simulink model "Vejlupek_CAR4_dsPIC33_AxleControl_bckup_R091228_R02"  (Simulink 7.3)
settings: Solver=FixedStepDiscrete  StartTime=0.0  StopTime=10.0  FixedStep=0.001  RelTol=1e-3
libraries: dsPICdrivers x14
settings Model: Creator=Bobes  LastModifiedBy=Bobes
settings OptimizationCC: OptimizeModelRefInitCode=on  LifeSpan=1
settings HardwareCC: ProdBitPerInt=16  ProdEndianess=LittleEndian  ProdWordSize=16  ProdHWDeviceType=16-bit Generic
settings RTWCC: SystemTargetFile=dspic.tlc  TemplateMakefile=dspic_pic30_gcc.tmf  PostCodeGenCommand=dsPIC_Compile()  Description=Embedded Target for Microchip dsPIC (real-time)  ProcessScript=dspic_make_rtw_hook
settings CodeAppCC: IgnoreCustomStorageClasses=off
settings STFCustomTargetCC: ModelReferenceCompliant=off  IncludeMdlTerminateFcn=off  CombineOutputUpdateFcns=on  SuppressErrorStatus=on  ERTCustomFileBanners=on  SupportContinuousTime=off  SupportNonInlinedSFcns=off  SystemTargetFile=dspic.tlc
settings ERTTargetCC: MultiwordLength=2048  ModelReferenceCompliant=off  ParMdlRefBuildCompliant=off  CompOptLevelCompliant=off  IncludeMdlTerminateFcn=off  SuppressErrorStatus=on  ERTFirstTimeCompliant=off  ModelStepFunctionPrototypeControlCompliant=off  CPPClassGenCompliant=off  InlinedParameterPlacement=NonHierarchical  ERTSrcFileBannerTemplate=dsPIC_code_template.cgt  ERTHdrFileBannerTemplate=dsPIC_code_template.cgt  ERTDataSrcFileTemplate=dsPIC_code_template.cgt  ERTDataHdrFileTemplate=dsPIC_code_template.cgt  ERTCustomFileTemplate=dsPIC_main.tlc
settings CustomProperty: DataType=string  Value=C:\PROGRA~1\MATLAB\R2009a\bin\win32\gmake

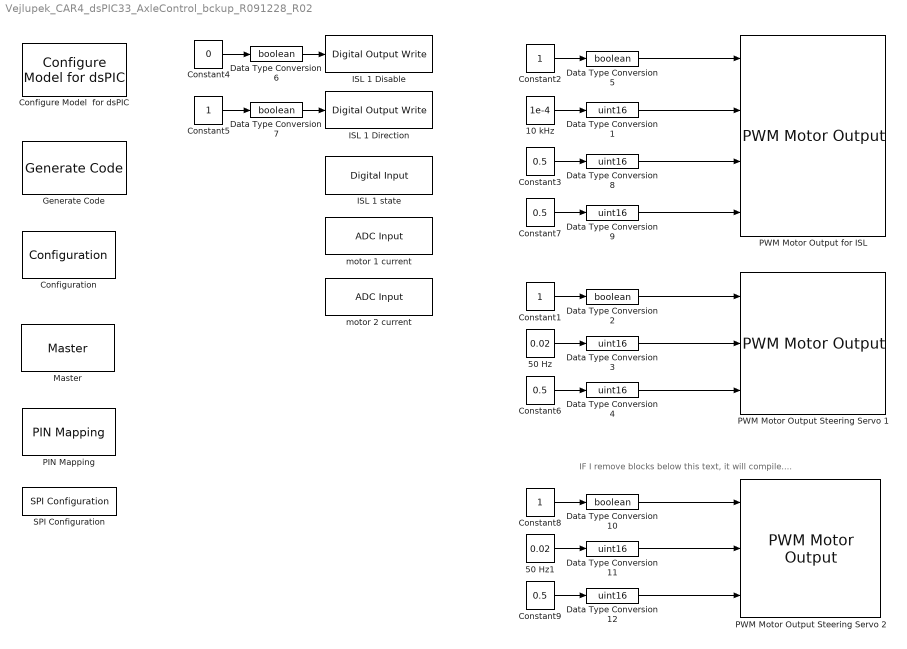
== system Vejlupek_CAR4_dsPIC33_AxleControl_bckup_R091228_R02 ==
  note: IF I remove blocks below this text, it will compile....
  10 kHz : Constant  Value=1e-4  OutDataType=fixdt(1, 16)  OutScaling=2^0
  50 Hz : Constant  Value=0.02  OutDataType=fixdt(1, 16)  OutScaling=2^0
  50 Hz1 : Constant  Value=0.02  OutDataType=fixdt(1, 16)  OutScaling=2^0
  Configuration : dsPICdrivers/Configuration  SystemSampleTime=-1  double64=on
  Configure Model  for dsPIC : dsPICdrivers/Simulink Configuration/Configure Model  for dsPIC
  Constant1 : Constant  OutDataType=fixdt(1, 16)  OutScaling=2^0
  Constant2 : Constant  OutDataType=fixdt(1, 16)  OutScaling=2^0
  Constant{3,6..7,9} (4 alike) : Constant  Value=0.5  OutDataType=fixdt(1, 16)  OutScaling=2^0
  Constant4 : Constant  Value=0  OutDataTypeMode=boolean  OutDataType=fixdt(1, 16)  OutScaling=2^0  OutDataTypeStr=boolean
  Constant5 : Constant  OutDataTypeMode=boolean  OutDataType=fixdt(1, 16)  OutScaling=2^0  OutDataTypeStr=boolean
  Constant8 : Constant  OutDataType=fixdt(1, 16)  OutScaling=2^0
  Data Type Conversion{1,3..4,8..9,11..12} (7 alike) : DataTypeConversion  OutDataTypeMode=uint16  OutDataType=fixdt(1, 16)  OutScaling=2^0  OutDataTypeStr=uint16
  Data Type Conversion{2,5..7,10} (5 alike) : DataTypeConversion  OutDataTypeMode=boolean  OutDataType=fixdt(1, 16)  OutScaling=2^0  OutDataTypeStr=boolean
  Generate Code : dsPICdrivers/Simulink Configuration/Generate Code
  ISL 1 Direction : dsPICdrivers/Digital I//O/Digital Output Write  Tag=dsPIC_Digital_Output  Priority=5  PORT=B  Pin=[4]  Simultaneous=off  OrderingInOutPopup=None
  ISL 1 Disable : dsPICdrivers/Digital I//O/Digital Output Write  Tag=dsPIC_Digital_Output  Priority=5  PORT=B  Pin=[3]  Simultaneous=off  OrderingInOutPopup=None
  ISL 1 state : dsPICdrivers/Digital I//O/Digital Input  Tag=dsPIC_Digital_Input  PORT=B  Pin=[2]  SampleTime=-1  OrderingInOutPopup=None
  Master : dsPICdrivers/Master  Tag=dsPIC_MASTER  Priority=1  TimeStepType=Timer1  picType=33fj128MC802  fcy=20000000  Quartz_33f=40e6  PLLActive_33f=off  fcyDesired_33f=20e6  tmr1="[1  19999  0]"  tmr1Info="Time Step : 0.001  ;   Error : 0%  PR1=19999"  tmr2345="[0  0  0  0]"  tmr2345cfg=[-1 -1 -1 -1]  IOautoConf=on  typePort="[ 8   8   0   0   0   0   0   0   0   0   0   0   0   0   0   0  22  22   9  10  10   0   0   0   0   0   0   0   0   0   0   0   0   0   0   0   0   0   0   0   0   0   0   0   0   0   0   0   0   0   0   0   0   0   0   0   0   0   0   0   0   0   0   0   0   0   0   0   0   0   0   0   0   0   0   0   0   0   0   0   0   0   0   0   0   0   0   0   0   0   0   0   0   0   0   0   0   0   0   0   0   0   0   0   0   0   0   0   0   0   0   0 ]"  TRIS="[ 65535  65511  65535  65535  65535  65535  65535 ]"  ADPCFG=60  MasterBusyPort=None  MasterOverloadPort=None  FOSC=External Clock  ClockSwitchMonitor=Both disabled  TempProtection_33f=TEMP_ON  FPBOR=<empty>  PWRT=disable  MCLR=<empty>  PowerSave=off  OverrideFcy=off  NewFcy=1e6  PR2345="[65535  65535  65535  65535]"
  PIN Mapping : dsPICdrivers/Peripheral MAPPING/PIN Mapping  Tag=dsPIC_PIN_Mapping  in_INT1=Not tied (VSS)  in_INT2=Not tied (VSS)  in_T2CK=Not tied (VSS)  in_T3CK=Not tied (VSS)  in_T4CK=Not tied (VSS)  in_T5CK=Not tied (VSS)  in_IC1=Not tied (VSS)  in_IC2=Not tied (VSS)  in_IC7=Not tied (VSS)  in_IC8=Not tied (VSS)  out_OC1=Not changed  out_OC2=Not changed  out_OC3=Not changed  out_OC4=Not changed  in_OCFA=Not tied (VSS)  in_FLTA1=Not tied (VSS)  in_FLTA2=Not tied (VSS)  in_QEA1=tied to RP0  in_QEB1=tied to RP1  in_INDX1=Not tied (VSS)  out_UPDN1=Not changed  out_UPDN2=Not changed  in_QEA2=Not changed  in_QEB2=Not changed  in_INDX2=Not tied (VSS)  in_U1RX=Not tied (VSS)  out_U1TX=Not changed  in_U1CTS=Not tied (VSS)  out_U1RTS=Not changed  in_U2RX=Not tied (VSS)  out_U2TX=Not changed  in_U2CTS=Not tied (VSS)  out_U2RTS=Not changed  in_SDI1=Not tied (VSS)  out_SDO1=Not changed  in_SCK1=Not tied (VSS)  out_SCK1OUT=Not changed  in_SS1=Not tied (VSS)  out_SS1OUT=Not changed  in_SDI2=Not tied (VSS)  out_SDO2=Not changed  in_SCK2=Not tied (VSS)  out_SCK2OUT=Not changed  in_SS2=Not tied (VSS)  out_SS2OUT=Not changed  in_C1RX=Not changed  out_C1TX=Not changed  out_C1OUT=Not changed  out_C2OUT=Not changed
  PWM Motor Output Steering Servo 1 : dsPICdrivers/Peripheral I//O/PWM Motor Output  Tag=dsPIC_PWM_Motor  Priority=5  PWMref=1  PWM12=2  InputEnableChk=on  InputPeriodeChk=on  Channel=[3]  TPeriode=0.02  PrescalerValue=16  PeriodeInteger=25000  MaxName='PWM'  Centered=off  HChannelON=off  Info="Nbr Bits : 15.6096  ||  PWM = 50000  ||  Prescaler = 16"  Delay=0  IntPriority=5  nbrPwmChannelPIC=3  Status=OK  DeadTimePrescaleA=0  DeadTimePrescaleB=0  DeadTimeInfo="Dead Time A = 0  ||  Dead Time B = 0"  DTPWM1a=Prescaler A  DTPWM1i=Prescaler A  DTPWM2a=Prescaler A  DTPWM2i=Prescaler A  DTPWM3a=Prescaler A  DTPWM3i=Prescaler A  DTPWM4a=Prescaler A  DTPWM4i=Prescaler A  DTCON1=0  DTCON2=0
  PWM Motor Output Steering Servo 2 : dsPICdrivers/Peripheral I//O/PWM Motor Output  Tag=dsPIC_PWM_Motor  Priority=5  PWMref=2  PWM12=2  InputEnableChk=on  InputPeriodeChk=on  Channel=[1]  TPeriode=.02  PrescalerValue=16  PeriodeInteger=25000  MaxName='PWM'  Centered=off  HChannelON=off  Info="Nbr Bits : 15.6096  ||  PWM = 50000  ||  Prescaler = 16"  Delay=0  IntPriority=5  nbrPwmChannelPIC=1  Status=OK  DeadTimePrescaleA=0  DeadTimePrescaleB=0  DeadTimeInfo="Dead Time A = 0  ||  Dead Time B = 0"  DTPWM1a=Prescaler A  DTPWM1i=Prescaler A  DTPWM2a=Prescaler A  DTPWM2i=Prescaler A  DTPWM3a=Prescaler A  DTPWM3i=Prescaler A  DTPWM4a=Prescaler A  DTPWM4i=Prescaler A  DTCON1=0  DTCON2=0
  PWM Motor Output for ISL : dsPICdrivers/Peripheral I//O/PWM Motor Output  Tag=dsPIC_PWM_Motor  Priority=5  PWMref=1  PWM12=2  InputEnableChk=on  InputPeriodeChk=on  Channel=[1 2]  TPeriode=1e-5  PrescalerValue=1  PeriodeInteger=200  MaxName='PWM'  Centered=off  HChannelON=off  Info="Nbr Bits : 8.6439  ||  PWM = 400  ||  Prescaler = 1"  Delay=0  IntPriority=5  nbrPwmChannelPIC=3  Status=OK  DeadTimePrescaleA=0  DeadTimePrescaleB=0  DeadTimeInfo="Dead Time A = 0  ||  Dead Time B = 0"  DTPWM1a=Prescaler A  DTPWM1i=Prescaler A  DTPWM2a=Prescaler A  DTPWM2i=Prescaler A  DTPWM3a=Prescaler A  DTPWM3i=Prescaler A  DTPWM4a=Prescaler A  DTPWM4i=Prescaler A  DTCON1=0  DTCON2=0
  SPI Configuration : dsPICdrivers/SPI PORT/SPI Configuration  Tag=dsPIC_config_SPI  Priority=2  ConfigurationTime=At boot time (only once)  OrderingInOutPopup=None  SampleTime=-1  Frame_Enable=0  Frame_Sync=None  SPI=1  MODE=MASTER  USER_SCALER=20  StartEnable=Enable  SDO_EN=off  DATA_LENGTH=16 bits  SS_EN=off  SMP=End of bit  CKP=high  CKE=Idle to Active  Status="OK - Mode 1  -    Fsck= 1000000Hz"
  motor 1 current : dsPICdrivers/Peripheral I//O/ADC Input  Tag=dsPIC_ADC  Priority=5  ADC_TYPE=10 bits  ADC_MODE=Continuous sampling & get last channel value  NbrSampleStep=1  VoltRefpopup="AVdd  -  AVss"  OutFormatBitspopup=0000 00dd dddd dddd : Integer  InterruptPriority=6  ANCHANNELS=[0]  MaxName=ANmax = 1023  Rin=1e2  ADCS=6  SAMC=1  Temperature=25  DMAChannel=0  SampleTime=-1  Status="OK  |  Tsmp=1.750e-007 |  T/Channel=2.275e-006 |  Tall=2.275e-006"  SSRC=auto convert
  motor 2 current : dsPICdrivers/Peripheral I//O/ADC Input  Tag=dsPIC_ADC  Priority=5  ADC_TYPE=10 bits  ADC_MODE=Continuous sampling & get last channel value  NbrSampleStep=1  VoltRefpopup="AVdd  -  AVss"  OutFormatBitspopup=0000 00dd dddd dddd : Integer  InterruptPriority=6  ANCHANNELS=[1]  MaxName=ANmax = 1023  Rin=1e2  ADCS=6  SAMC=1  Temperature=25  DMAChannel=0  SampleTime=-1  Status="OK  |  Tsmp=1.750e-007 |  T/Channel=2.275e-006 |  Tall=2.275e-006"  SSRC=auto convert
  wires:
  Constant2/1 -> Data Type Conversion5/1
  Data Type Conversion5/1 -> PWM Motor Output for ISL/1
  Constant1/1 -> Data Type Conversion2/1
  Data Type Conversion2/1 -> PWM Motor Output Steering Servo 1/1
  Data Type Conversion3/1 -> PWM Motor Output Steering Servo 1/2
  Data Type Conversion4/1 -> PWM Motor Output Steering Servo 1/3
  10 kHz/1 -> Data Type Conversion1/1
  Data Type Conversion1/1 -> PWM Motor Output for ISL/2
  50 Hz/1 -> Data Type Conversion3/1
  Constant6/1 -> Data Type Conversion4/1
  Constant5/1 -> Data Type Conversion7/1
  Data Type Conversion7/1 -> ISL 1 Direction/1
  Constant4/1 -> Data Type Conversion6/1
  Data Type Conversion6/1 -> ISL 1 Disable/1
  Constant3/1 -> Data Type Conversion8/1
  Constant7/1 -> Data Type Conversion9/1
  Data Type Conversion8/1 -> PWM Motor Output for ISL/3
  Data Type Conversion9/1 -> PWM Motor Output for ISL/4
  Constant8/1 -> Data Type Conversion10/1
  50 Hz1/1 -> Data Type Conversion11/1
  Constant9/1 -> Data Type Conversion12/1
  Data Type Conversion10/1 -> PWM Motor Output Steering Servo 2/1
  Data Type Conversion11/1 -> PWM Motor Output Steering Servo 2/2
  Data Type Conversion12/1 -> PWM Motor Output Steering Servo 2/3
